simulink model "homework13"  (R2023b)
settings: Solver=VariableStepAuto  StartTime=0.0  StopTime=inf  RelTol=1e-3
libraries: ros2lib x2, simulink x1
settings Model: Creator=hby  LastModifiedBy=hby

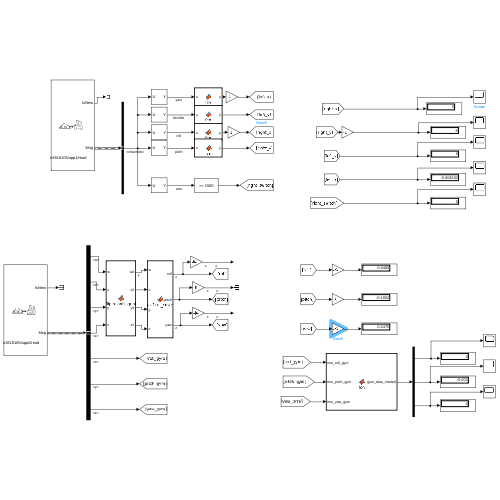
[thumbnail: Simulink's stored preview of the top-level diagram]
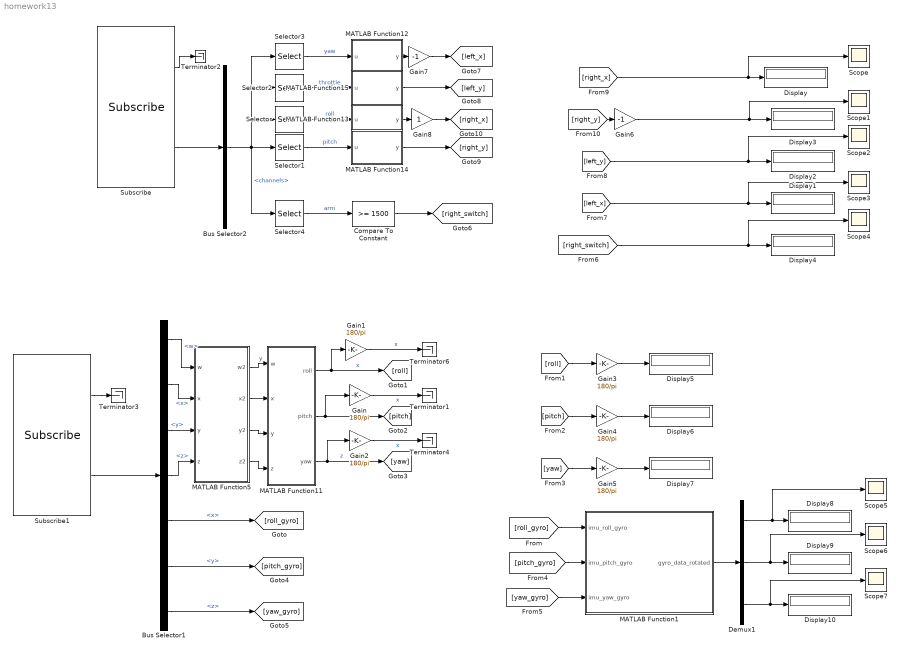
== system homework13 ==
  Bus Selector1 : BusSelector  OutputSignals=orientation.w,orientation.x,orientation.y,orientation.z,angular_velocity.x,angular_velocity.y,angular_velocity.z
  Bus Selector2 : BusSelector  OutputSignals=channels
  Compare To Constant : simulink/Logic and Bit Operations/Compare To Constant  relop=>=  const=1500  OutDataTypeStr=boolean
  Demux1 : Demux  Outputs=3
  Display{,1..10} (11 alike) : Display
  Gain{,1..5} (6 alike) : Gain  Gain=180/pi
  Gain6 : Gain  Gain=-1
  Gain7 : Gain  Gain=-1
  Gain8 : Gain
  MATLAB Function1 : MATLAB Function  TreatAsAtomicUnit=on
  MATLAB Function11 : MATLAB Function  TreatAsAtomicUnit=on
  MATLAB Function12 : MATLAB Function  TreatAsAtomicUnit=on
  MATLAB Function13 : MATLAB Function  TreatAsAtomicUnit=on
  MATLAB Function14 : MATLAB Function  TreatAsAtomicUnit=on
  MATLAB Function15 : MATLAB Function  TreatAsAtomicUnit=on
  MATLAB Function5 : MATLAB Function  TreatAsAtomicUnit=on
  Scope{,1..7} (8 alike) : Scope
  Selector : Selector  InputPortWidth=128  IndexOptions=Index vector (dialog)  Indices=1  OutputSizes=1
  Selector1 : Selector  InputPortWidth=128  IndexOptions=Index vector (dialog)  Indices=2  OutputSizes=1
  Selector2 : Selector  InputPortWidth=128  IndexOptions=Index vector (dialog)  Indices=3  OutputSizes=1
  Selector3 : Selector  InputPortWidth=128  IndexOptions=Index vector (dialog)  Indices=4  OutputSizes=1
  Selector4 : Selector  InputPortWidth=128  IndexOptions=Index vector (dialog)  Indices=6  OutputSizes=1
  Subscribe : ros2lib/Subscribe  topicSource=Select from ROS network  topic=/ecat/sn2818105/app1/read  messageType=custom_msgs/ReadSBUSRC  sampleTime=-1  QOSHistory=Keep last  QOSDepth=1  QOSReliability=Best effort  QOSDurability=Volatile
  Subscribe1 : ros2lib/Subscribe  topicSource=Select from ROS network  topic=/ecat/sn2818105/app2/read  messageType=sensor_msgs/Imu  sampleTime=-1  QOSHistory=Keep last  QOSDepth=1  QOSReliability=Best effort  QOSDurability=Volatile
  Terminator{1..4,6} (5 alike) : Terminator
  wires:
  Gain8/1 -> [right_x]
  Subscribe/2 -> Bus Selector2/1
  MATLAB Function12/1(y) -> Gain7/1
  [right_y] -> Gain6/1
  Bus Selector2/1 -> Selector4/1, Selector1/1, Selector3/1, Selector2/1, Selector/1  "<channels>"
  Selector1/1 -> MATLAB Function14/1(u)  "pitch"
  MATLAB Function14/1(y) -> [right_y]
  Selector/1 -> MATLAB Function13/1(u)  "roll"
  Selector3/1 -> MATLAB Function12/1(u)  "yaw"
  [right_x] -> Scope/1, Display/1
  Selector2/1 -> MATLAB Function15/1(u)  "throttle"
  MATLAB Function13/1(y) -> Gain8/1
  Subscribe/1 -> Terminator2/1
  Compare To Constant/1 -> [right_switch]
  MATLAB Function15/1(y) -> [left_y]
  Selector4/1 -> Compare To Constant/1  "arm"
  Gain7/1 -> [left_x]
  Gain6/1 -> Scope1/1, Display3/1
  [left_y] -> Scope2/1, Display2/1
  [left_x] -> Scope3/1, Display1/1
  [right_switch] -> Scope4/1, Display4/1
  MATLAB Function5/4(z2) -> MATLAB Function11/4(z)
  MATLAB Function11/2(pitch) -> [pitch], Gain/1
  MATLAB Function11/3(yaw) -> Gain2/1, [yaw]  "z"
  Bus Selector1/5 -> [roll_gyro]  "<x>"
  MATLAB Function11/1(roll) -> Gain1/1, [roll]  "x"
  MATLAB Function5/2(x2) -> MATLAB Function11/2(x)
  MATLAB Function5/3(y2) -> MATLAB Function11/3(y)
  Bus Selector1/4 -> MATLAB Function5/4(z)  "<z>"
  MATLAB Function5/1(w2) -> MATLAB Function11/1(w)  "y"
  Bus Selector1/1 -> MATLAB Function5/1(w)  "<w>"
  Subscribe1/2 -> Bus Selector1/1
  Bus Selector1/3 -> MATLAB Function5/3(y)  "<y>"
  Bus Selector1/2 -> MATLAB Function5/2(x)  "<x>"
  Subscribe1/1 -> Terminator3/1
  Bus Selector1/7 -> [yaw_gyro]  "<z>"
  Bus Selector1/6 -> [pitch_gyro]  "<y>"
  Gain1/1 -> Terminator6/1  "x"
  Gain/1 -> Terminator1/1  "x"
  Gain2/1 -> Terminator4/1  "x"
  [roll] -> Gain3/1
  [pitch] -> Gain4/1
  [yaw] -> Gain5/1
  [pitch_gyro] -> MATLAB Function1/2(imu_pitch_gyro)
  [yaw_gyro] -> MATLAB Function1/3(imu_yaw_gyro)
  MATLAB Function1/1(gyro_data_rotated) -> Demux1/1
  [roll_gyro] -> MATLAB Function1/1(imu_roll_gyro)
  Demux1/1 -> Scope5/1, Display8/1
  Demux1/2 -> Scope6/1, Display9/1
  Demux1/3 -> Scope7/1, Display10/1
  Gain3/1 -> Display5/1
  Gain4/1 -> Display6/1
  Gain5/1 -> Display7/1

== matlab function homework13/MATLAB Function1 ==
  data: imu_roll_gyro input; gyro_data_rotated output; imu_pitch_gyro input; imu_yaw_gyro input
function gyro_data_rotated = fcn(imu_roll_gyro, imu_pitch_gyro, imu_yaw_gyro)

% 定义角速度向量
gyro_data = [imu_roll_gyro; imu_pitch_gyro; imu_yaw_gyro];

% 定义绕 x 轴旋转 180 度的旋转矩阵
xy_flip_matrix = [1  0  0;
                  0 -1  0;
                  0  0 -1];

% 应用旋转矩阵
gyro_data_rotated = xy_flip_matrix* gyro_data;

== matlab function homework13/MATLAB Function5 ==
  data: w input; w2 output; x input; y input; z input; x2 output; y2 output; z2 output
function [w2, x2, y2, z2] = flip_x_axis_quat(w, x, y, z)
% 输入: 四元数(w, x, y, z), x向右y向前z向上
% 输出: 四元数(w2, x2, y2, z2), x反向(y/z不变)

% 四元数转旋转矩阵
R = quat2rotm([w x y z]);

% x轴取反变换矩阵
Mx = [-1 0 0;
       0 1 0;
       0 0 1];

% 应用镜像变换
R_flip = Mx * R * Mx;

% 旋转矩阵转回四元数
q2 = rotm2quat(R_flip);

% 保证四元数为标准形式
if q2(1)<0
    q2 = -q2;
end

% 输出
w2 = q2(1);
x2 = q2(2);
y2 = q2(3);
z2 = q2(4);
end

function R = quat2rotm(q)
% 四元数 -> 旋转矩阵，q=[w x y z]
w = q(1); x = q(2); y = q(3); z = q(4);
R = [1-2*(y^2+z^2), 2*(x*y-w*z),   2*(x*z+w*y);
     2*(x*y+w*z),   1-2*(x^2+z^2), 2*(y*z-w*x);
     2*(x*z-w*y),   2*(y*z+w*x),   1-2*(x^2+y^2)];
end

function q = rotm2quat(R)
% 旋转矩阵 -> 四元数，输出q=[w x y z]
tr = trace(R);
if tr > 0
    S = sqrt(tr+1.0)*2; % S=4*qw
    qw = 0.25*S;
    qx = (R(3,2)-R(2,3))/S;
    qy = (R(1,3)-R(3,1))/S;
    qz = (R(2,1)-R(1,2))/S;
elseif (R(1,1) > R(2,2)) && (R(1,1) > R(3,3))
    S = sqrt(1.0+R(1,1)-R(2,2)-R(3,3))*2;
    qw = (R(3,2)-R(2,3))/S;
    qx = 0.25*S;
    qy = (R(1,2)+R(2,1))/S;
    qz = (R(1,3)+R(3,1))/S;
elseif (R(2,2) > R(3,3))
    S = sqrt(1.0+R(2,2)-R(1,1)-R(3,3))*2;
    qw = (R(1,3)-R(3,1))/S;
    qx = (R(1,2)+R(2,1))/S;
    qy = 0.25*S;
    qz = (R(2,3)+R(3,2))/S;
else
    S = sqrt(1.0+R(3,3)-R(1,1)-R(2,2))*2;
    qw = (R(2,1)-R(1,2))/S;
    qx = (R(1,3)+R(3,1))/S;
    qy = (R(2,3)+R(3,2))/S;
    qz = 0.25*S;
end
q = [qw qx qy qz];
end

== matlab function homework13/MATLAB Function11 ==
  data: w input; roll output; x input; y input; z input; pitch output; yaw output
function [roll, pitch, yaw] = quat2eul_custom(w, x, y, z)
% 输入: w, x, y, z 四元数
% 输出: roll, pitch, yaw (ZYX顺序，单位：弧度)

q = [w, x, y, z];

% 计算欧拉角 (ZYX顺序)
yaw = atan2(2*(w*z + x*y), 1 - 2*(y^2 + z^2));
pitch = asin(2*(w*y - z*x));
roll = atan2(2*(w*x + y*z), 1 - 2*(x^2 + y^2));
end

== matlab function homework13/MATLAB Function12 ==
  data: u input; y output
function y = fcn(u)

RC_MIN = 341;
RC_MID = 1024;
RC_MAX = 1706;
DEADZONE = 20;

u = double(u);

if u > RC_MID + DEADZONE
    y = (u - RC_MID - DEADZONE) / ...
        (RC_MAX - RC_MID - DEADZONE);

elseif u < RC_MID - DEADZONE
    y = (u - RC_MID + DEADZONE) / ...
        (RC_MID - RC_MIN - DEADZONE);

else
    y = 0;
end

% 限幅
if y > 1
    y = 1;
elseif y < -1
    y = -1;
end

== matlab function homework13/MATLAB Function13 ==
  data: u input; y output
function y = fcn(u)

RC_MIN = 341;
RC_MID = 1024;
RC_MAX = 1706;
DEADZONE = 20;

u = double(u);

if u > RC_MID + DEADZONE
    y = (u - RC_MID - DEADZONE) / ...
        (RC_MAX - RC_MID - DEADZONE);

elseif u < RC_MID - DEADZONE
    y = (u - RC_MID + DEADZONE) / ...
        (RC_MID - RC_MIN - DEADZONE);

else
    y = 0;
end

% 限幅
if y > 1
    y = 1;
elseif y < -1
    y = -1;
end

== matlab function homework13/MATLAB Function14 ==
  data: u input; y output
function y = fcn(u)

RC_MIN = 341;
RC_MID = 1024;
RC_MAX = 1706;
DEADZONE = 20;

u = double(u);

if u > RC_MID + DEADZONE
    y = (u - RC_MID - DEADZONE) / ...
        (RC_MAX - RC_MID - DEADZONE);

elseif u < RC_MID - DEADZONE
    y = (u - RC_MID + DEADZONE) / ...
        (RC_MID - RC_MIN - DEADZONE);

else
    y = 0;
end

% 限幅
if y > 1
    y = 1;
elseif y < -1
    y = -1;
end

== matlab function homework13/MATLAB Function15 ==
  data: u input; y output
function y = fcn(u)

RC_MIN = 341;
RC_MID = 1024;
RC_MAX = 1706;
DEADZONE = 20;

u = double(u);

if u > RC_MID + DEADZONE
    y = (u - RC_MID - DEADZONE) / ...
        (RC_MAX - RC_MID - DEADZONE);

elseif u < RC_MID - DEADZONE
    y = (u - RC_MID + DEADZONE) / ...
        (RC_MID - RC_MIN - DEADZONE);

else
    y = 0;
end

% 限幅
if y > 1
    y = 1;
elseif y < -1
    y = -1;
end
